simulink library "blocksLibrary"  (R2024b)
settings: Solver=VariableStepAuto  StartTime=0.0  StopTime=10.0  RelTol=1e-3
values from neighbouring files (symbols this model uses):
  maxWaypoints = 20    [createVariables.m]
undefined symbols (not defined in the file or in its folder): gen3
settings Model: Creator=scastro  LastModifiedBy=esaro
settings SolverCC: AlgebraicLoopSolver=TrustRegion
settings DataIOCC: ReturnWorkspaceOutputs=off
settings DebuggingCC: UnconnectedInputMsg=warning  UnconnectedOutputMsg=warning  UnconnectedLineMsg=warning  PregeneratedLibrarySubsystemCodeDiagnostic=none  ArithmeticOperatorsInVariantConditions=warning
settings ModelReferenceCC: EnableRefExpFcnMdlSchedulingChecks=on
settings SFSimCC: SimUseLocalCustomCode=off  CustomCodeUndefinedFunction=UseInterfaceOnly
settings RTWCC: RTWUseLocalCustomCode=off  GPUComputeCapability=3.5

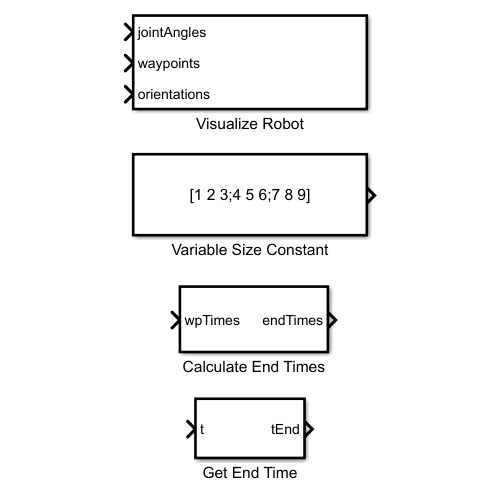
[thumbnail: Simulink's stored preview of the top-level diagram]
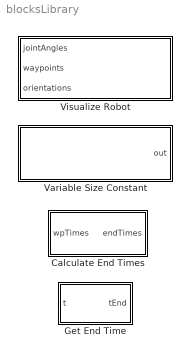
== system blocksLibrary ==
  Calculate End Times : MATLAB Function  TreatAsAtomicUnit=on  mask(Calculate End Times){maxSize=maxWaypoints, trajDof=3}
      mask prompts: maxSize "Maximum Number of Waypoints"; trajDof "Trajectory Degrees of Freedom"
      mask help: Accepts a vector of waypoint times and calculates end times for trapezoidal trajectories
  Get End Time : MATLAB Function  TreatAsAtomicUnit=on  mask(Get End Time){maxWaypoints=maxWaypoints}
      mask prompts: maxWaypoints "Maximum Number of Waypoints"
      mask help: Gets end time from an array of times.
  Variable Size Constant : MATLAB Function  TreatAsAtomicUnit=on  mask(Variable Size Constant){val=[1 2 3;4 5 6;7 8 9], maxSize=[20, 3], Ts=-1}
      mask prompts: val "Value"; maxSize "Maximum Size"; Ts "Output Sample Time"
      mask help: Creates a variable-size constant (up to 2D)
  Visualize Robot : MATLAB Function  InitFcn=clear visualizeRobot;  TreatAsAtomicUnit=on  mask(Visualize Robot){rbtName=gen3, eeName=Gripper, numJoints=numel(gen3.homeConfiguration), maxPts=maxWaypoints, plotMode=Trajectory}
      mask prompts: rbtName "Rigid Body Tree Name"; eeName "End Effector Name"; numJoints "Number of Joints"; maxPts "Max Number of Waypoints"; plotMode "Plot Mode"
      mask help: Displays a Rigid Body Tree, its waypoints, and end effector trajectory.

== matlab function blocksLibrary/Visualize Robot ==
  data: jointAngles input size=numJoints; waypoints input size=[3,maxPts]; orientations input size=[3,maxPts]; plotMode parameter
function showRobot(jointAngles,waypoints,orientations,plotMode)
% Wrapper function that visualizes the robot in simulation.
       
    % Extract rigid body tree and end effector names from the block dialog
    coder.extrinsic('gcb');
    coder.extrinsic('get_param');
    persistent rbtName eeName
    if isempty(rbtName)
       rbtName = get_param(gcb,'rbtName'); 
       eeName = get_param(gcb,'eeName'); 
    end
    
    coder.extrinsic('visualizeRobot'); % Will be ignored for code generation
    visualizeRobot(rbtName,eeName,jointAngles,waypoints,orientations,plotMode);

end

== matlab function blocksLibrary/Calculate End Times ==
  data: wpTimes input size=[1 maxSize]; endTimes output size=[trajDof maxSize-1]; trajDof parameter
function endTimes = calcEndTimes(wpTimes, trajDof)

% Calculate trajectory segment end times from waypoint time vector,
% and replicate the rows based on the DOFs of the trajectory.
endTimes = repmat(diff(wpTimes),[trajDof 1]);

== matlab function blocksLibrary/Get End Time ==
  data: t input size=[1 maxWaypoints]; tEnd output
function tEnd = getEnd(t)

if ~isempty(t)
    tEnd = t(end);
else
    tEnd = 0;
end

== matlab function blocksLibrary/Variable Size Constant ==
  settings: updateMethod=DISCRETE  sampleTime=Ts
  data: out output size=maxSize; val parameter
function out = varSizeConst(val)
% Creates a variable-size constant (up to 2D)

out = val;

end
